simulink model "FlexibleDriveLineTestHarness"  (R2025b)
settings: Solver=daessc  StartTime=0.0  StopTime=10.0  FixedStep=0.0001  RelTol=1e-3
PreLoadFcn:
  | FlexibleDriveLineTestHarnessParams;
undefined symbols (not defined in the file or in its folder): thParams
libraries: fl_lib x5, nesl_utility x2, simulink x1
settings Model: Creator=shachind  LastModifiedBy=shachind
settings SimscapeCC: SimscapeLogType=all  SimscapeLogName=simlogMechanicalDLTorsion

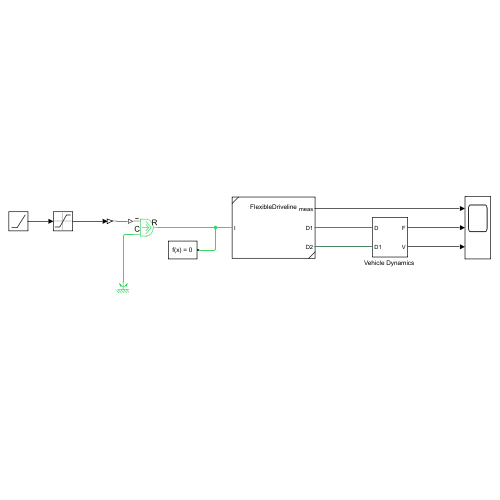
[thumbnail: Simulink's stored preview of the top-level diagram]
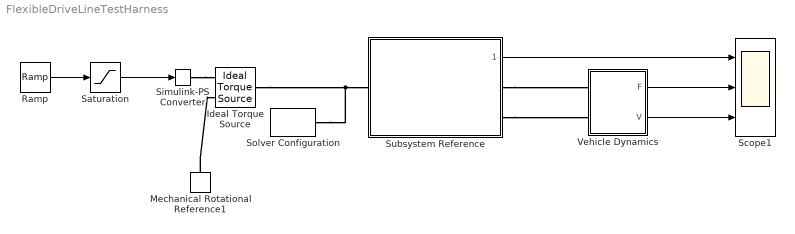
== system FlexibleDriveLineTestHarness ==
  Ideal Torque Source : fl_lib/Mechanical/Mechanical Sources/Ideal Torque Source
  Mechanical Rotational Reference1 : fl_lib/Mechanical/Rotational Elements/Mechanical Rotational Reference
  Ramp : simulink/Sources/Ramp  slope=thParams.ramp.slope  start=0.01  InitialOutput=0
  Saturation : Saturate  UpperLimit=thParams.saturation.upperLimit  LowerLimit=thParams.saturation.lowerLimit
  Scope1 : Scope  NumInputPorts=3
      settings: ActiveDisplayYMinimum=-122.32922095817939  ActiveDisplayYMaximum=303.22554705884659
  Simulink-PS Converter : nesl_utility/Simulink-PS Converter  PhysicalDomain=network_engine_domain  SubClassName=ps_input  LeftPortType=input  RightPortType=output  PseudoPeriodic=off  Frequencies=[]  NoiseDistribution=none  NoiseParameters=[]  Unit=1  AffineConversion=off  FilteringAndDerivatives=provide  SimscapeFilterOrder=1  InputFilterTimeConstant=0.001  UdotUserProvided=0
  Solver Configuration : nesl_utility/Solver Configuration  PhysicalDomain=network_engine_domain  SubClassName=solver  LeftPortType=input  RightPortType=generic  Tones=[]  Harmonics=[]  SimulateNoise=off  Profile=off  UseLocalSampling=off  EnableSwitchedLinearOptims=on  FrequencyDomain=off  UseCCode=off  RelTol=0.001  AbsTol=0.001  MinStep=1e-09  ToWorkspace=off  RevertToSquareIcSolve=off  NumHomotopyIterations=100  PhasorMode=off  PhasorModeNumHarmonics=1  ConsistencySolver=NEWTON_XTOL_AFTER_FTOL  IndexReductionMethod=DerivativeReplacement  DoDC=off  ResidualTolerance=1e-09  ConsistencyTolSource=GLOBAL  ConsistencyAbsTol=0.001  ConsistencyRelTol=0.001  ConsistencyTolFactor=0.001  UseLocalSolver=on  LocalSolverChoice=NE_BACKWARD_EULER_ADVANCER  ResolveIndetEquations=on  FunctionEvalNumThread=1  LocalSolverSampleTime=0.0001  DoFixedCost=off  MaxNonlinIter=3  MaxModeIter=2  ComputeImpulses=off  ImpulseIterations=2  LinearAlgebra=auto  LinearAlgebraNumThread=0  EquationFormulation=NE_TIME_EF  DelaysMemoryBudget=1024  AutomaticFiltering=on  FilteringTimeConstant=0.001  PartitionStorageMethod=AS_NEEDED  PartitionMemoryBudget=1024  PartitionMethod=ROBUST  MultibodyUseLocalSolver=off  MultibodyLocalSolverChoice=ODE1  MultibodyLocalSolverSampleTime=0.001
  Subsystem Reference : Subsystem  ReferencedSubsystem=FlexibleDriveline
  "Vehicle Dynamics " : Subsystem
  wires:
  "Vehicle Dynamics "/1(F) -> Scope1/2
  "Vehicle Dynamics "/2(V) -> Scope1/3
  Saturation/1 -> Simulink-PS Converter/1
  Ramp/1 -> Saturation/1
  Subsystem Reference/1 -> Scope1/1
  connections:
  Subsystem Reference/RConn1 -- "Vehicle Dynamics "/LConn1
  Ideal Torque Source/LConn1 -- Solver Configuration/RConn1 -- Subsystem Reference/LConn1
  Simulink-PS Converter/RConn1 -- Ideal Torque Source/RConn1
  Mechanical Rotational Reference1/LConn1 -- Ideal Torque Source/RConn2
  Subsystem Reference/RConn2 -- "Vehicle Dynamics "/LConn2

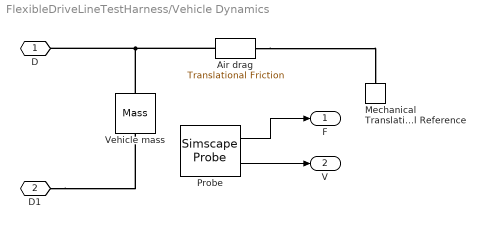
== system FlexibleDriveLineTestHarness/Vehicle Dynamics  ==
  "Air drag " : fl_lib/Mechanical/Translational Elements/Translational Friction  brkwy_frc=300 N  brkwy_vel=0.01 m/s  Col_frc=150 N  visc_coef=1000 N*s/m  v_specify=off  v_priority=None  v=0 m/s  v_nominal_specify=off  v_nominal_value=1  v_nominal_unit=m/s  f_specify=off  f_priority=None  f=0 N  f_nominal_specify=off  f_nominal_value=1  f_nominal_unit=N
      settings: InternalSimscapePortConfiguration="{\"Bottom\":[],\"Left\":[{\"id\":\"R\",\"label\":\"R\",\"type\":\"foundation.mechanical.translational.translational\"}],\"Right\":[{\"id\":\"C\",\"label\":\"C\",\"type\":\"foundation.mechanical.translational.translational\"}],\"Top\":[]}"
  Mechanical Translational Reference : fl_lib/Mechanical/Translational Elements/Mechanical Translational Reference
  Probe : SimscapeProbe  BoundBlock=50  Variables="{\"f\":{\"Probing\":\"ON\"},\"v\":{\"Probing\":\"ON\"}}"
  Vehicle mass : fl_lib/Mechanical/Translational Elements/Mass  mass=thParams.vehicle.mass kg  num_ports=foundation.enum.numPorts2.two  v_specify=off  v_priority=High  v=0 m/s  v_nominal_specify=off  v_nominal_value=1  v_nominal_unit=m/s  f_specify=off  f_priority=None  f=0 N  f_nominal_specify=off  f_nominal_value=1  f_nominal_unit=N
      settings: InternalSimscapePortConfiguration="{\"Bottom\":[],\"Left\":[{\"id\":\"M\",\"label\":\"\",\"type\":\"foundation.mechanical.translational.translational\"}],\"Right\":[{\"id\":\"N\",\"label\":\"\",\"type\":\"foundation.mechanical.translational.translational\"}],\"Top\":[]}"
  D : PMIOPort  Side=Left
  D1 : PMIOPort  Port=2  Side=Left
  F : Outport
  V : Outport  Port=2
  wires:
  Probe/1 -> F/1
  Probe/2 -> V/1
  connections:
  "Air drag "/RConn1 -- Mechanical Translational Reference/LConn1
  "Air drag "/LConn1 -- Vehicle mass/LConn1 -- D/RConn1
  D1/RConn1 -- Vehicle mass/RConn1
